simulink model "sparrow_albatros_spec_withgpio"  (R2021a)
settings: Solver=VariableStepDiscrete  StartTime=0.0  StopTime=100  RelTol=1e-3
undefined symbols (not defined in the file): pfb_coeff_gen_calc
libraries: xbsIndex_r4 x5582, casper_library_misc x33, casper_library_delays x28, xps_library x10, simulink x8, xbsReplacements_r4 x2
(part 31 of 80)

== system sparrow_albatros_spec_withgpio/fft_wideband_real/fft_biplex_real_4x/biplex_core/fft_stage_6 ==
  in1 : Inport
  in2 : Inport  Port=2
  of_in : Inport  Port=3
  sync : Inport  Port=4
  shift : Inport  Port=5
  butterfly_direct : Subsystem  AncestorBlock=casper_library_ffts/butterfly_direct  mask(butterfly_direct){n_inputs=1, biplex=on, FFTSize=FFTSize, Coeffs=[0 1 2 3 4 5 6 7 8 9 10 11 12 13 14 15 16 17 18 19 20 21 22 23 24 25 26 27 28 29 30 31], StepPeriod=5, coeff_bit_width=coeff_bit_width, input_bit_width=input_bit_width, bin_pt_in=bin_pt_in, downshift=off, async=off, floating_point=off, float_type=single, exp_width=8, frac_width=24, add_latency=add_latency, mult_latency=mult_latency, bram_latency=bram_latency, conv_latency=conv_latency, add_pipe_latency=0, mult_pipe_latency=0, quantization=Round  (unbiased: Even Values), overflow=Saturate, coeffs_bit_limit=coeffs_bit_limit, coeff_sharing=on, coeff_decimation=on, coeff_generation=off, cal_bits=1, n_bits_rotation=25, max_fanout=max_fanout, use_hdl=on, use_embedded=off, bitgrowth=on, hardcode_shifts=off, dsp48_adders=off}
      mask prompts: n_inputs "number inputs"; biplex "Used in biplex FFT"; FFTSize "Size of FFT: (2^? pts)"; Coeffs "Coefficients: (0 to 2^(FFTSize-1)-1)"; StepPeriod "Coefficient Step Period: (2^?)"; coeff_bit_width "Coefficient Bit Width"; input_bit_width "Input Bit Width"; bin_pt_in "Input binary point"; async "asynchronous operation"; floating_point "floating point"; float_type "float type"; exp_width "exponent width"; frac_width "fraction width"; add_latency "Add Latency"; mult_latency "Mult Latency"; bram_latency "BRAM Latency"; conv_latency "Convert latency"; add_pipe_latency "Add Pipeline Latency"; mult_pipe_latency "Mult Pipeline Latency"; quantization "Quantization Behavior"; overflow "Overflow Behavior"; coeffs_bit_limit "Number bits above which to store stage's coefficients in BRAM (2^? bits)"; coeff_sharing "BRAM sharing in coeff storage"; coeff_decimation "Store a fraction of coeff factors where useful"; coeff_generation "Generate coeffs with multipliers where useful"; cal_bits "Number calibration locations when generating coeffs (2^?)"; n_bits_rotation "Feedback rotation vector resolution"; max_fanout "Maximum fanout"; use_hdl "Use behavioural HDL for multipliers"; use_embedded "Use embedded multipliers"; bitgrowth "Bit growth instead of shifting"; hardcode_shifts "Hardcode shift schedule"; dsp48_adders "Use DSP48s for adders"
      mask help: FFT internal block.
      mask init: same as sparrow_albatros_spec_withgpio/fft_wideband_real/fft_direct/butterfly0_0
      settings: AttributesFormatString=twiddle_general
      mask Callback floating_point:
      | onoff = get_param(gcb, 'floating_point');
      | if strcmp(onoff,'on')
      |     enable_fixpt = 'off';
      |     set_param_state(gcb, 'float_type', 'on')
      | 
      |     f_type = get_param(gcb, 'float_type');
      |     if strcmp(f_type,'custom')
      |         set_param_state(gcb, 'exp_width', 'on')
      |         set_param_state(gcb, 'frac_width', 'on')
      |     else
      |         set_param_state(gcb, 'exp_width', 'off')
      |         set_param_state(gcb, 'frac_width', 'off')
      |     end
      | 
      | 
      | else
      |     enable_fixpt = 'on';
      |     set_param_state(gcb, 'float_type', 'off')
      |     set_param_state(gcb, 'exp_width', 'off')
      |     set_param_state(gcb, 'frac_width', 'off')
      | end
      | 
      | set_param_state(gcb, 'input_bit_width', enable_fixpt)
      | set_param_state(gcb, 'bin_pt_in', enable_fixpt)
      | set_param_state(gcb, 'coeff_bit_width', enable_fixpt)
      mask TypeOptions float_type: single | custom
      mask Callback float_type:
      | f_type = get_param(gcb, 'float_type');
      | if strcmp(f_type,'custom')
      |     set_param_state(gcb, 'exp_width', 'on')
      |     set_param_state(gcb, 'frac_width', 'on')
      | else
      |     set_param_state(gcb, 'exp_width', 'off')
      |     set_param_state(gcb, 'frac_width', 'off')
      | end
      mask TypeOptions quantization: Truncate | Round  (unbiased: +/- Inf) | Round  (unbiased: Even Values)
      mask TypeOptions overflow: Wrap | Saturate | Error
      mask Callback use_hdl:
      | % make mutually exclusive with use_embedded.
      | 
      | use_hdl = get_param(gcb, 'use_hdl');
      | if strcmp(use_hdl, 'on'),
      |     set_param_state(gcb, 'use_embedded', 'off');
      | else
      |     set_param_state(gcb, 'use_embedded', 'on');
      | end
      mask Callback use_embedded:
      | % make mutually exclusive with use_hdl.
      | 
      | use_hdl = get_param(gcb, 'use_embedded');
      | if strcmp(use_hdl, 'on'),
      |     set_param_state(gcb, 'use_hdl', 'off');
      | else
      |     set_param_state(gcb, 'use_hdl', 'on');
      | end
      mask Callback hardcode_shifts:
      | hardcode_shifts = get_param(gcb, 'hardcode_shifts');
      | set_param_state(gcb, 'downshift', hardcode_shifts);
      mask Callback dsp48_adders: %fft_callback_dsp48_adders(gcb);
      mask DialogControl ParameterTabVar0 Prompt: Basic
      mask DialogControl ParameterTabVar01 Prompt: Latency
      mask DialogControl ParameterTabVar012 Prompt: Implementation
  counter : xbsIndex_r4/Counter  cnt_type=Free Running  cnt_to=Inf  operation=Up  start_count=0  cnt_by_val=1  arith_type=Unsigned  n_bits=FFTSize-FFTStage+1  bin_pt=0  load_pin=off  rst=on  en=off  explicit_period=on  period=1  use_behavioral_HDL=off  implementation=Fabric  dbl_ovrd=off  block_type=counter
  delay0 : Subsystem  AncestorBlock=casper_library_bus/bus_delay  mask(bus_delay){n_bits=23, csp_latency=2^(FFTSize-FFTStage), cmplx=on, enable=off, reg_retiming=on, misc=off}
      mask prompts: n_bits "input bit widths"; csp_latency "latency"; cmplx "complex data"; enable "enable port"; reg_retiming "implement using behavioral HDL"; misc "misc support"
      mask help: Delay components of a bus
      mask init:
      | bus_delay_init(gcb, ...
      |     'enable', enable, ...
      |     'cmplx', cmplx, ...
      |     'n_bits', n_bits, ...
      |     'csp_latency', csp_latency, ...
      |     'reg_retiming', reg_retiming, ...
      |     'misc', misc);
  delay1 : Subsystem  AncestorBlock=casper_library_bus/bus_delay  mask(bus_delay){n_bits=23, csp_latency=2^(FFTSize-FFTStage), cmplx=on, enable=off, reg_retiming=on, misc=off}
      mask prompts: n_bits "input bit widths"; csp_latency "latency"; cmplx "complex data"; enable "enable port"; reg_retiming "implement using behavioral HDL"; misc "misc support"
      mask help: Delay components of a bus
      mask init:
      | bus_delay_init(gcb, ...
      |     'enable', enable, ...
      |     'cmplx', cmplx, ...
      |     'n_bits', n_bits, ...
      |     'csp_latency', csp_latency, ...
      |     'reg_retiming', reg_retiming, ...
      |     'misc', misc);
  din0 : xbsIndex_r4/Delay  rst=off  infoeditControl=Selection of Reset will increase slice count due to use of real FFs and instead of SRLs  en=off  latency=0  reg_retiming=on  dbl_ovrd=off  block_type=delay
  din2 : xbsIndex_r4/Delay  rst=off  infoeditControl=Selection of Reset will increase slice count due to use of real FFs and instead of SRLs  en=off  latency=0  reg_retiming=on  dbl_ovrd=off  block_type=delay
  dmux0 : xbsIndex_r4/Delay  rst=off  infoeditControl=Selection of Reset will increase slice count due to use of real FFs and instead of SRLs  en=off  latency=0  reg_retiming=on  dbl_ovrd=off  block_type=delay
  dmux1 : xbsIndex_r4/Delay  rst=off  infoeditControl=Selection of Reset will increase slice count due to use of real FFs and instead of SRLs  en=off  latency=0  reg_retiming=on  dbl_ovrd=off  block_type=delay
  dsync0 : xbsIndex_r4/Delay  rst=off  infoeditControl=Selection of Reset will increase slice count due to use of real FFs and instead of SRLs  en=off  latency=0  reg_retiming=on  dbl_ovrd=off  block_type=delay
  dsync1 : xbsIndex_r4/Delay  rst=off  infoeditControl=Selection of Reset will increase slice count due to use of real FFs and instead of SRLs  en=off  latency=1  reg_retiming=on  dbl_ovrd=off  block_type=delay
  logical1 : xbsIndex_r4/Logical  logical_function=OR  inputs=2  en=off  latency=1  precision=Full  arith_type=Unsigned  n_bits=16  bin_pt=0  align_bp=on  dbl_ovrd=off  block_type=logical
  mux0 : xbsIndex_r4/Mux  inputs=2  en=off  latency=1  precision=Full  arith_type=Unsigned  n_bits=16  bin_pt=14  quantization=Truncate  overflow=Wrap  dbl_ovrd=off  block_type=mux
  mux1 : xbsIndex_r4/Mux  inputs=2  en=off  latency=1  precision=Full  arith_type=Unsigned  n_bits=16  bin_pt=14  quantization=Truncate  overflow=Wrap  dbl_ovrd=off  block_type=mux
  slice0 : xbsIndex_r4/Slice  nbits=1  boolean_output=on  mode=Lower Bit Location + Width  bit1=-(FFTStage - 1)  base1=MSB of Input  bit0=FFTStage - 1  base0=LSB of Input  dbl_ovrd=off  block_type=slice
  slice1 : xbsIndex_r4/Slice  nbits=1  boolean_output=off  mode=Upper Bit Location + Width  bit1=0  base1=MSB of Input  bit0=0  base0=LSB of Input  dbl_ovrd=off  block_type=slice
  sync_delay : casper_library_delays/sync_delay  DelayLen=2^(FFTSize - FFTStage)
      settings: SourceProductName=CASPER DSP Blockset
  out1 : Outport
  out2 : Outport  Port=2
  of : Outport  Port=3
  sync_out : Outport  Port=4
  wires:
  in1/1 -> din0/1
  sync/1 -> dsync0/1
  counter/1 -> slice1/1
  slice1/1 -> mux1/1, mux0/1
  mux0/1 -> dmux0/1
  din0/1 -> mux1/2, mux0/3
  dsync0/1 -> dsync1/1, counter/1
  in2/1 -> din2/1
  din2/1 -> delay0/1(din)
  mux1/1 -> dmux1/1
  dmux1/1 -> delay1/1(din)
  delay0/1(dout) -> mux1/3, mux0/2
  dsync1/1 -> sync_delay/1
  shift/1 -> slice0/1
  dmux0/1 -> butterfly_direct/2(b)
  slice0/1 -> butterfly_direct/4(shift)
  delay1/1(dout) -> butterfly_direct/1(a)
  sync_delay/1 -> butterfly_direct/3(sync_in)
  of_in/1 -> logical1/2
  butterfly_direct/3(of) -> logical1/1
  butterfly_direct/1(a+bw) -> out1/1
  butterfly_direct/2(a-bw) -> out2/1
  logical1/1 -> of/1
  butterfly_direct/4(sync_out) -> sync_out/1

== system sparrow_albatros_spec_withgpio/fft_wideband_real/fft_biplex_real_4x/biplex_core/fft_stage_7 ==
  in1 : Inport
  in2 : Inport  Port=2
  of_in : Inport  Port=3
  sync : Inport  Port=4
  shift : Inport  Port=5
  butterfly_direct : Subsystem  AncestorBlock=casper_library_ffts/butterfly_direct  mask(butterfly_direct){n_inputs=1, biplex=on, FFTSize=FFTSize, Coeffs=[0 1 2 3 4 5 6 7 8 9 10 11 12 13 14 15 16 17 18 19 20 21 22 23 24 25 26 27 28 29 30 31 32 33 34 35 36 37 38 39 40 41 42 43 44 45 46 47 48 49 50 51 52 53 54 55 56 57 58 59 60 61 62 63], StepPeriod=4, coeff_bit_width=coeff_bit_width, input_bit_width=input_bit_width, bin_pt_in=bin_pt_in, downshift=off, async=off, floating_point=off, float_type=single, exp_width=8, frac_width=24, add_latency=add_latency, mult_latency=mult_latency, bram_latency=bram_latency, conv_latency=conv_latency, add_pipe_latency=0, mult_pipe_latency=0, quantization=Round  (unbiased: Even Values), overflow=Saturate, coeffs_bit_limit=coeffs_bit_limit, coeff_sharing=on, coeff_decimation=on, coeff_generation=off, cal_bits=1, n_bits_rotation=25, max_fanout=max_fanout, use_hdl=on, use_embedded=off, bitgrowth=off, hardcode_shifts=off, dsp48_adders=off}
      mask prompts: n_inputs "number inputs"; biplex "Used in biplex FFT"; FFTSize "Size of FFT: (2^? pts)"; Coeffs "Coefficients: (0 to 2^(FFTSize-1)-1)"; StepPeriod "Coefficient Step Period: (2^?)"; coeff_bit_width "Coefficient Bit Width"; input_bit_width "Input Bit Width"; bin_pt_in "Input binary point"; async "asynchronous operation"; floating_point "floating point"; float_type "float type"; exp_width "exponent width"; frac_width "fraction width"; add_latency "Add Latency"; mult_latency "Mult Latency"; bram_latency "BRAM Latency"; conv_latency "Convert latency"; add_pipe_latency "Add Pipeline Latency"; mult_pipe_latency "Mult Pipeline Latency"; quantization "Quantization Behavior"; overflow "Overflow Behavior"; coeffs_bit_limit "Number bits above which to store stage's coefficients in BRAM (2^? bits)"; coeff_sharing "BRAM sharing in coeff storage"; coeff_decimation "Store a fraction of coeff factors where useful"; coeff_generation "Generate coeffs with multipliers where useful"; cal_bits "Number calibration locations when generating coeffs (2^?)"; n_bits_rotation "Feedback rotation vector resolution"; max_fanout "Maximum fanout"; use_hdl "Use behavioural HDL for multipliers"; use_embedded "Use embedded multipliers"; bitgrowth "Bit growth instead of shifting"; hardcode_shifts "Hardcode shift schedule"; dsp48_adders "Use DSP48s for adders"
      mask help: FFT internal block.
      mask init: same as sparrow_albatros_spec_withgpio/fft_wideband_real/fft_direct/butterfly0_0
      settings: AttributesFormatString=twiddle_general
      mask Callback floating_point:
      | onoff = get_param(gcb, 'floating_point');
      | if strcmp(onoff,'on')
      |     enable_fixpt = 'off';
      |     set_param_state(gcb, 'float_type', 'on')
      | 
      |     f_type = get_param(gcb, 'float_type');
      |     if strcmp(f_type,'custom')
      |         set_param_state(gcb, 'exp_width', 'on')
      |         set_param_state(gcb, 'frac_width', 'on')
      |     else
      |         set_param_state(gcb, 'exp_width', 'off')
      |         set_param_state(gcb, 'frac_width', 'off')
      |     end
      | 
      | 
      | else
      |     enable_fixpt = 'on';
      |     set_param_state(gcb, 'float_type', 'off')
      |     set_param_state(gcb, 'exp_width', 'off')
      |     set_param_state(gcb, 'frac_width', 'off')
      | end
      | 
      | set_param_state(gcb, 'input_bit_width', enable_fixpt)
      | set_param_state(gcb, 'bin_pt_in', enable_fixpt)
      | set_param_state(gcb, 'coeff_bit_width', enable_fixpt)
      mask TypeOptions float_type: single | custom
      mask Callback float_type:
      | f_type = get_param(gcb, 'float_type');
      | if strcmp(f_type,'custom')
      |     set_param_state(gcb, 'exp_width', 'on')
      |     set_param_state(gcb, 'frac_width', 'on')
      | else
      |     set_param_state(gcb, 'exp_width', 'off')
      |     set_param_state(gcb, 'frac_width', 'off')
      | end
      mask TypeOptions quantization: Truncate | Round  (unbiased: +/- Inf) | Round  (unbiased: Even Values)
      mask TypeOptions overflow: Wrap | Saturate | Error
      mask Callback use_hdl:
      | % make mutually exclusive with use_embedded.
      | 
      | use_hdl = get_param(gcb, 'use_hdl');
      | if strcmp(use_hdl, 'on'),
      |     set_param_state(gcb, 'use_embedded', 'off');
      | else
      |     set_param_state(gcb, 'use_embedded', 'on');
      | end
      mask Callback use_embedded:
      | % make mutually exclusive with use_hdl.
      | 
      | use_hdl = get_param(gcb, 'use_embedded');
      | if strcmp(use_hdl, 'on'),
      |     set_param_state(gcb, 'use_hdl', 'off');
      | else
      |     set_param_state(gcb, 'use_hdl', 'on');
      | end
      mask Callback hardcode_shifts:
      | hardcode_shifts = get_param(gcb, 'hardcode_shifts');
      | set_param_state(gcb, 'downshift', hardcode_shifts);
      mask Callback dsp48_adders: %fft_callback_dsp48_adders(gcb);
      mask DialogControl ParameterTabVar0 Prompt: Basic
      mask DialogControl ParameterTabVar01 Prompt: Latency
      mask DialogControl ParameterTabVar012 Prompt: Implementation
  counter : xbsIndex_r4/Counter  cnt_type=Free Running  cnt_to=Inf  operation=Up  start_count=0  cnt_by_val=1  arith_type=Unsigned  n_bits=FFTSize-FFTStage+1  bin_pt=0  load_pin=off  rst=on  en=off  explicit_period=on  period=1  use_behavioral_HDL=off  implementation=Fabric  dbl_ovrd=off  block_type=counter
  delay0 : Subsystem  AncestorBlock=casper_library_bus/bus_delay  mask(bus_delay){n_bits=24, csp_latency=2^(FFTSize-FFTStage), cmplx=on, enable=off, reg_retiming=on, misc=off}
      mask prompts: n_bits "input bit widths"; csp_latency "latency"; cmplx "complex data"; enable "enable port"; reg_retiming "implement using behavioral HDL"; misc "misc support"
      mask help: Delay components of a bus
      mask init:
      | bus_delay_init(gcb, ...
      |     'enable', enable, ...
      |     'cmplx', cmplx, ...
      |     'n_bits', n_bits, ...
      |     'csp_latency', csp_latency, ...
      |     'reg_retiming', reg_retiming, ...
      |     'misc', misc);
  delay1 : Subsystem  AncestorBlock=casper_library_bus/bus_delay  mask(bus_delay){n_bits=24, csp_latency=2^(FFTSize-FFTStage), cmplx=on, enable=off, reg_retiming=on, misc=off}
      mask prompts: n_bits "input bit widths"; csp_latency "latency"; cmplx "complex data"; enable "enable port"; reg_retiming "implement using behavioral HDL"; misc "misc support"
      mask help: Delay components of a bus
      mask init:
      | bus_delay_init(gcb, ...
      |     'enable', enable, ...
      |     'cmplx', cmplx, ...
      |     'n_bits', n_bits, ...
      |     'csp_latency', csp_latency, ...
      |     'reg_retiming', reg_retiming, ...
      |     'misc', misc);
  din0 : xbsIndex_r4/Delay  rst=off  infoeditControl=Selection of Reset will increase slice count due to use of real FFs and instead of SRLs  en=off  latency=0  reg_retiming=on  dbl_ovrd=off  block_type=delay
  din2 : xbsIndex_r4/Delay  rst=off  infoeditControl=Selection of Reset will increase slice count due to use of real FFs and instead of SRLs  en=off  latency=0  reg_retiming=on  dbl_ovrd=off  block_type=delay
  dmux0 : xbsIndex_r4/Delay  rst=off  infoeditControl=Selection of Reset will increase slice count due to use of real FFs and instead of SRLs  en=off  latency=0  reg_retiming=on  dbl_ovrd=off  block_type=delay
  dmux1 : xbsIndex_r4/Delay  rst=off  infoeditControl=Selection of Reset will increase slice count due to use of real FFs and instead of SRLs  en=off  latency=0  reg_retiming=on  dbl_ovrd=off  block_type=delay
  dsync0 : xbsIndex_r4/Delay  rst=off  infoeditControl=Selection of Reset will increase slice count due to use of real FFs and instead of SRLs  en=off  latency=0  reg_retiming=on  dbl_ovrd=off  block_type=delay
  dsync1 : xbsIndex_r4/Delay  rst=off  infoeditControl=Selection of Reset will increase slice count due to use of real FFs and instead of SRLs  en=off  latency=1  reg_retiming=on  dbl_ovrd=off  block_type=delay
  logical1 : xbsIndex_r4/Logical  logical_function=OR  inputs=2  en=off  latency=1  precision=Full  arith_type=Unsigned  n_bits=16  bin_pt=0  align_bp=on  dbl_ovrd=off  block_type=logical
  mux0 : xbsIndex_r4/Mux  inputs=2  en=off  latency=1  precision=Full  arith_type=Unsigned  n_bits=16  bin_pt=14  quantization=Truncate  overflow=Wrap  dbl_ovrd=off  block_type=mux
  mux1 : xbsIndex_r4/Mux  inputs=2  en=off  latency=1  precision=Full  arith_type=Unsigned  n_bits=16  bin_pt=14  quantization=Truncate  overflow=Wrap  dbl_ovrd=off  block_type=mux
  slice0 : xbsIndex_r4/Slice  nbits=1  boolean_output=on  mode=Lower Bit Location + Width  bit1=-(FFTStage - 1)  base1=MSB of Input  bit0=FFTStage - 1  base0=LSB of Input  dbl_ovrd=off  block_type=slice
  slice1 : xbsIndex_r4/Slice  nbits=1  boolean_output=off  mode=Upper Bit Location + Width  bit1=0  base1=MSB of Input  bit0=0  base0=LSB of Input  dbl_ovrd=off  block_type=slice
  sync_delay : casper_library_delays/sync_delay  DelayLen=2^(FFTSize - FFTStage)
      settings: SourceProductName=CASPER DSP Blockset
  out1 : Outport
  out2 : Outport  Port=2
  of : Outport  Port=3
  sync_out : Outport  Port=4
  wires:
  in1/1 -> din0/1
  sync/1 -> dsync0/1
  counter/1 -> slice1/1
  slice1/1 -> mux1/1, mux0/1
  mux0/1 -> dmux0/1
  din0/1 -> mux1/2, mux0/3
  dsync0/1 -> dsync1/1, counter/1
  in2/1 -> din2/1
  din2/1 -> delay0/1(din)
  mux1/1 -> dmux1/1
  dmux1/1 -> delay1/1(din)
  delay0/1(dout) -> mux1/3, mux0/2
  dsync1/1 -> sync_delay/1
  shift/1 -> slice0/1
  dmux0/1 -> butterfly_direct/2(b)
  slice0/1 -> butterfly_direct/4(shift)
  delay1/1(dout) -> butterfly_direct/1(a)
  sync_delay/1 -> butterfly_direct/3(sync_in)
  of_in/1 -> logical1/2
  butterfly_direct/3(of) -> logical1/1
  butterfly_direct/1(a+bw) -> out1/1
  butterfly_direct/2(a-bw) -> out2/1
  logical1/1 -> of/1
  butterfly_direct/4(sync_out) -> sync_out/1

== system sparrow_albatros_spec_withgpio/fft_wideband_real/fft_biplex_real_4x/biplex_core/fft_stage_8 ==
  in1 : Inport
  in2 : Inport  Port=2
  of_in : Inport  Port=3
  sync : Inport  Port=4
  shift : Inport  Port=5
  butterfly_direct : Subsystem  AncestorBlock=casper_library_ffts/butterfly_direct  mask(butterfly_direct){n_inputs=1, biplex=on, FFTSize=FFTSize, Coeffs=[0 1 2 3 4 5 6 7 8 9 10 11 12 13 14 15 16 17 18 19 20 21 22 23 24 25 26 27 28 29 30 31 32 33 34 35 36 37 38 39 40 41 42 43 44 45 46 47 48 49 50 51 52 53 54 55 56 57 58 59 60 61 62 63 64 65 66 67 68 69 70 71 72 73 74 75 76 77 78 79 80 81 82 83 84 85 86 87 88 89 90 91 92 93 94 95 96 97 98 99 100 101 102 103 104 105 106 107 108 109 110 111 112 113 114 115 116 117 118 119 120 121 122 123 124 125 126 127], StepPeriod=3, coeff_bit_width=coeff_bit_width, input_bit_width=input_bit_width, bin_pt_in=bin_pt_in, downshift=off, async=off, floating_point=off, float_type=single, exp_width=8, frac_width=24, add_latency=add_latency, mult_latency=mult_latency, bram_latency=bram_latency, conv_latency=conv_latency, add_pipe_latency=0, mult_pipe_latency=0, quantization=Round  (unbiased: Even Values), overflow=Saturate, coeffs_bit_limit=coeffs_bit_limit, coeff_sharing=on, coeff_decimation=on, coeff_generation=off, cal_bits=1, n_bits_rotation=25, max_fanout=max_fanout, use_hdl=on, use_embedded=off, bitgrowth=off, hardcode_shifts=off, dsp48_adders=off}
      mask prompts: n_inputs "number inputs"; biplex "Used in biplex FFT"; FFTSize "Size of FFT: (2^? pts)"; Coeffs "Coefficients: (0 to 2^(FFTSize-1)-1)"; StepPeriod "Coefficient Step Period: (2^?)"; coeff_bit_width "Coefficient Bit Width"; input_bit_width "Input Bit Width"; bin_pt_in "Input binary point"; async "asynchronous operation"; floating_point "floating point"; float_type "float type"; exp_width "exponent width"; frac_width "fraction width"; add_latency "Add Latency"; mult_latency "Mult Latency"; bram_latency "BRAM Latency"; conv_latency "Convert latency"; add_pipe_latency "Add Pipeline Latency"; mult_pipe_latency "Mult Pipeline Latency"; quantization "Quantization Behavior"; overflow "Overflow Behavior"; coeffs_bit_limit "Number bits above which to store stage's coefficients in BRAM (2^? bits)"; coeff_sharing "BRAM sharing in coeff storage"; coeff_decimation "Store a fraction of coeff factors where useful"; coeff_generation "Generate coeffs with multipliers where useful"; cal_bits "Number calibration locations when generating coeffs (2^?)"; n_bits_rotation "Feedback rotation vector resolution"; max_fanout "Maximum fanout"; use_hdl "Use behavioural HDL for multipliers"; use_embedded "Use embedded multipliers"; bitgrowth "Bit growth instead of shifting"; hardcode_shifts "Hardcode shift schedule"; dsp48_adders "Use DSP48s for adders"
      mask help: FFT internal block.
      mask init: same as sparrow_albatros_spec_withgpio/fft_wideband_real/fft_direct/butterfly0_0
      settings: AttributesFormatString=twiddle_general
      mask Callback floating_point:
      | onoff = get_param(gcb, 'floating_point');
      | if strcmp(onoff,'on')
      |     enable_fixpt = 'off';
      |     set_param_state(gcb, 'float_type', 'on')
      | 
      |     f_type = get_param(gcb, 'float_type');
      |     if strcmp(f_type,'custom')
      |         set_param_state(gcb, 'exp_width', 'on')
      |         set_param_state(gcb, 'frac_width', 'on')
      |     else
      |         set_param_state(gcb, 'exp_width', 'off')
      |         set_param_state(gcb, 'frac_width', 'off')
      |     end
      | 
      | 
      | else
      |     enable_fixpt = 'on';
      |     set_param_state(gcb, 'float_type', 'off')
      |     set_param_state(gcb, 'exp_width', 'off')
      |     set_param_state(gcb, 'frac_width', 'off')
      | end
      | 
      | set_param_state(gcb, 'input_bit_width', enable_fixpt)
      | set_param_state(gcb, 'bin_pt_in', enable_fixpt)
      | set_param_state(gcb, 'coeff_bit_width', enable_fixpt)
      mask TypeOptions float_type: single | custom
      mask Callback float_type:
      | f_type = get_param(gcb, 'float_type');
      | if strcmp(f_type,'custom')
      |     set_param_state(gcb, 'exp_width', 'on')
      |     set_param_state(gcb, 'frac_width', 'on')
      | else
      |     set_param_state(gcb, 'exp_width', 'off')
      |     set_param_state(gcb, 'frac_width', 'off')
      | end
      mask TypeOptions quantization: Truncate | Round  (unbiased: +/- Inf) | Round  (unbiased: Even Values)
      mask TypeOptions overflow: Wrap | Saturate | Error
      mask Callback use_hdl:
      | % make mutually exclusive with use_embedded.
      | 
      | use_hdl = get_param(gcb, 'use_hdl');
      | if strcmp(use_hdl, 'on'),
      |     set_param_state(gcb, 'use_embedded', 'off');
      | else
      |     set_param_state(gcb, 'use_embedded', 'on');
      | end
      mask Callback use_embedded:
      | % make mutually exclusive with use_hdl.
      | 
      | use_hdl = get_param(gcb, 'use_embedded');
      | if strcmp(use_hdl, 'on'),
      |     set_param_state(gcb, 'use_hdl', 'off');
      | else
      |     set_param_state(gcb, 'use_hdl', 'on');
      | end
      mask Callback hardcode_shifts:
      | hardcode_shifts = get_param(gcb, 'hardcode_shifts');
      | set_param_state(gcb, 'downshift', hardcode_shifts);
      mask Callback dsp48_adders: %fft_callback_dsp48_adders(gcb);
      mask DialogControl ParameterTabVar0 Prompt: Basic
      mask DialogControl ParameterTabVar01 Prompt: Latency
      mask DialogControl ParameterTabVar012 Prompt: Implementation
  counter : xbsIndex_r4/Counter  cnt_type=Free Running  cnt_to=Inf  operation=Up  start_count=0  cnt_by_val=1  arith_type=Unsigned  n_bits=FFTSize-FFTStage+1  bin_pt=0  load_pin=off  rst=on  en=off  explicit_period=on  period=1  use_behavioral_HDL=off  implementation=Fabric  dbl_ovrd=off  block_type=counter
  delay0 : Subsystem  AncestorBlock=casper_library_bus/bus_delay  mask(bus_delay){n_bits=24, csp_latency=2^(FFTSize-FFTStage), cmplx=on, enable=off, reg_retiming=on, misc=off}
      mask prompts: n_bits "input bit widths"; csp_latency "latency"; cmplx "complex data"; enable "enable port"; reg_retiming "implement using behavioral HDL"; misc "misc support"
      mask help: Delay components of a bus
      mask init:
      | bus_delay_init(gcb, ...
      |     'enable', enable, ...
      |     'cmplx', cmplx, ...
      |     'n_bits', n_bits, ...
      |     'csp_latency', csp_latency, ...
      |     'reg_retiming', reg_retiming, ...
      |     'misc', misc);
  delay1 : Subsystem  AncestorBlock=casper_library_bus/bus_delay  mask(bus_delay){n_bits=24, csp_latency=2^(FFTSize-FFTStage), cmplx=on, enable=off, reg_retiming=on, misc=off}
      mask prompts: n_bits "input bit widths"; csp_latency "latency"; cmplx "complex data"; enable "enable port"; reg_retiming "implement using behavioral HDL"; misc "misc support"
      mask help: Delay components of a bus
      mask init:
      | bus_delay_init(gcb, ...
      |     'enable', enable, ...
      |     'cmplx', cmplx, ...
      |     'n_bits', n_bits, ...
      |     'csp_latency', csp_latency, ...
      |     'reg_retiming', reg_retiming, ...
      |     'misc', misc);
  din0 : xbsIndex_r4/Delay  rst=off  infoeditControl=Selection of Reset will increase slice count due to use of real FFs and instead of SRLs  en=off  latency=0  reg_retiming=on  dbl_ovrd=off  block_type=delay
  din2 : xbsIndex_r4/Delay  rst=off  infoeditControl=Selection of Reset will increase slice count due to use of real FFs and instead of SRLs  en=off  latency=0  reg_retiming=on  dbl_ovrd=off  block_type=delay
  dmux0 : xbsIndex_r4/Delay  rst=off  infoeditControl=Selection of Reset will increase slice count due to use of real FFs and instead of SRLs  en=off  latency=0  reg_retiming=on  dbl_ovrd=off  block_type=delay
  dmux1 : xbsIndex_r4/Delay  rst=off  infoeditControl=Selection of Reset will increase slice count due to use of real FFs and instead of SRLs  en=off  latency=0  reg_retiming=on  dbl_ovrd=off  block_type=delay
  dsync0 : xbsIndex_r4/Delay  rst=off  infoeditControl=Selection of Reset will increase slice count due to use of real FFs and instead of SRLs  en=off  latency=0  reg_retiming=on  dbl_ovrd=off  block_type=delay
  dsync1 : xbsIndex_r4/Delay  rst=off  infoeditControl=Selection of Reset will increase slice count due to use of real FFs and instead of SRLs  en=off  latency=1  reg_retiming=on  dbl_ovrd=off  block_type=delay
  logical1 : xbsIndex_r4/Logical  logical_function=OR  inputs=2  en=off  latency=1  precision=Full  arith_type=Unsigned  n_bits=16  bin_pt=0  align_bp=on  dbl_ovrd=off  block_type=logical
  mux0 : xbsIndex_r4/Mux  inputs=2  en=off  latency=1  precision=Full  arith_type=Unsigned  n_bits=16  bin_pt=14  quantization=Truncate  overflow=Wrap  dbl_ovrd=off  block_type=mux
  mux1 : xbsIndex_r4/Mux  inputs=2  en=off  latency=1  precision=Full  arith_type=Unsigned  n_bits=16  bin_pt=14  quantization=Truncate  overflow=Wrap  dbl_ovrd=off  block_type=mux
  slice0 : xbsIndex_r4/Slice  nbits=1  boolean_output=on  mode=Lower Bit Location + Width  bit1=-(FFTStage - 1)  base1=MSB of Input  bit0=FFTStage - 1  base0=LSB of Input  dbl_ovrd=off  block_type=slice
  slice1 : xbsIndex_r4/Slice  nbits=1  boolean_output=off  mode=Upper Bit Location + Width  bit1=0  base1=MSB of Input  bit0=0  base0=LSB of Input  dbl_ovrd=off  block_type=slice
  sync_delay : casper_library_delays/sync_delay  DelayLen=2^(FFTSize - FFTStage)
      settings: SourceProductName=CASPER DSP Blockset
  out1 : Outport
  out2 : Outport  Port=2
  of : Outport  Port=3
  sync_out : Outport  Port=4
  wires:
  in1/1 -> din0/1
  sync/1 -> dsync0/1
  counter/1 -> slice1/1
  slice1/1 -> mux1/1, mux0/1
  mux0/1 -> dmux0/1
  din0/1 -> mux1/2, mux0/3
  dsync0/1 -> dsync1/1, counter/1
  in2/1 -> din2/1
  din2/1 -> delay0/1(din)
  mux1/1 -> dmux1/1
  dmux1/1 -> delay1/1(din)
  delay0/1(dout) -> mux1/3, mux0/2
  dsync1/1 -> sync_delay/1
  shift/1 -> slice0/1
  dmux0/1 -> butterfly_direct/2(b)
  slice0/1 -> butterfly_direct/4(shift)
  delay1/1(dout) -> butterfly_direct/1(a)
  sync_delay/1 -> butterfly_direct/3(sync_in)
  of_in/1 -> logical1/2
  butterfly_direct/3(of) -> logical1/1
  butterfly_direct/1(a+bw) -> out1/1
  butterfly_direct/2(a-bw) -> out2/1
  logical1/1 -> of/1
  butterfly_direct/4(sync_out) -> sync_out/1

== system sparrow_albatros_spec_withgpio/fft_wideband_real/fft_biplex_real_4x/biplex_core/fft_stage_9 ==
  in1 : Inport
  in2 : Inport  Port=2
  of_in : Inport  Port=3
  sync : Inport  Port=4
  shift : Inport  Port=5
  butterfly_direct : Subsystem  AncestorBlock=casper_library_ffts/butterfly_direct  mask(butterfly_direct){n_inputs=1, biplex=on, FFTSize=FFTSize, Coeffs=[0 1 2 3 4 5 6 7 8 9 10 11 12 13 14 15 16 17 18 19 20 21 22 23 24 25 26 27 28 29 30 31 32 33 34 35 36 37 38 39 40 41 42 43 44 45 46 47 48 49 50 51 52 53 54 55 56 57 58 59 60 61 62 63 64 65 66 67 68 69 70 71 72 73 74 75 76 77 78 79 80 81 82 83 84 85 86 87 88 89 90 91 92 93 94 95 96 97 98 99 100 101 102 103 104 105 106 107 108 109 110 111 112 113 114 115 116 117 118 119 120 121 122 123 124 125 126 127 128 129 130 131 132 133 134 135 136 137 138 139 140 141 142 143 144 145 146 147 148 149 150 151 152 153 154 155 156 157 158 159 160 161 162 163 164 165 166 167 168 169 170 171 172 173 174 175 176 177 178 179 180 181 182 183 184 185 186 187 188 189 190 191 192 193 194 195 196 197 198 199 200 201 202 203 204 205 206 207 208 209 210 211 212 213 214 215 216 217 218 219 220 221 222 223 224 225 226 227 228 229 230 231 232 233 234 235 236 237 238 239 240 241 242 243 244 245 246 247 248 249 250 251 252 253 254 255], StepPeriod=2, coeff_bit_width=coeff_bit_width, input_bit_width=input_bit_width, bin_pt_in=bin_pt_in, downshift=off, async=off, floating_point=off, float_type=single, exp_width=8, frac_width=24, add_latency=add_latency, mult_latency=mult_latency, bram_latency=bram_latency, conv_latency=conv_latency, add_pipe_latency=0, mult_pipe_latency=0, quantization=Round  (unbiased: Even Values), overflow=Saturate, coeffs_bit_limit=coeffs_bit_limit, coeff_sharing=on, coeff_decimation=on, coeff_generation=off, cal_bits=1, n_bits_rotation=25, max_fanout=max_fanout, use_hdl=on, use_embedded=off, bitgrowth=off, hardcode_shifts=off, dsp48_adders=off}
      mask prompts: n_inputs "number inputs"; biplex "Used in biplex FFT"; FFTSize "Size of FFT: (2^? pts)"; Coeffs "Coefficients: (0 to 2^(FFTSize-1)-1)"; StepPeriod "Coefficient Step Period: (2^?)"; coeff_bit_width "Coefficient Bit Width"; input_bit_width "Input Bit Width"; bin_pt_in "Input binary point"; async "asynchronous operation"; floating_point "floating point"; float_type "float type"; exp_width "exponent width"; frac_width "fraction width"; add_latency "Add Latency"; mult_latency "Mult Latency"; bram_latency "BRAM Latency"; conv_latency "Convert latency"; add_pipe_latency "Add Pipeline Latency"; mult_pipe_latency "Mult Pipeline Latency"; quantization "Quantization Behavior"; overflow "Overflow Behavior"; coeffs_bit_limit "Number bits above which to store stage's coefficients in BRAM (2^? bits)"; coeff_sharing "BRAM sharing in coeff storage"; coeff_decimation "Store a fraction of coeff factors where useful"; coeff_generation "Generate coeffs with multipliers where useful"; cal_bits "Number calibration locations when generating coeffs (2^?)"; n_bits_rotation "Feedback rotation vector resolution"; max_fanout "Maximum fanout"; use_hdl "Use behavioural HDL for multipliers"; use_embedded "Use embedded multipliers"; bitgrowth "Bit growth instead of shifting"; hardcode_shifts "Hardcode shift schedule"; dsp48_adders "Use DSP48s for adders"
      mask help: FFT internal block.
      mask init: same as sparrow_albatros_spec_withgpio/fft_wideband_real/fft_direct/butterfly0_0
      settings: AttributesFormatString=twiddle_general
      mask Callback floating_point:
      | onoff = get_param(gcb, 'floating_point');
      | if strcmp(onoff,'on')
      |     enable_fixpt = 'off';
      |     set_param_state(gcb, 'float_type', 'on')
      | 
      |     f_type = get_param(gcb, 'float_type');
      |     if strcmp(f_type,'custom')
      |         set_param_state(gcb, 'exp_width', 'on')
      |         set_param_state(gcb, 'frac_width', 'on')
      |     else
      |         set_param_state(gcb, 'exp_width', 'off')
      |         set_param_state(gcb, 'frac_width', 'off')
      |     end
      | 
      | 
      | else
      |     enable_fixpt = 'on';
      |     set_param_state(gcb, 'float_type', 'off')
      |     set_param_state(gcb, 'exp_width', 'off')
      |     set_param_state(gcb, 'frac_width', 'off')
      | end
      | 
      | set_param_state(gcb, 'input_bit_width', enable_fixpt)
      | set_param_state(gcb, 'bin_pt_in', enable_fixpt)
      | set_param_state(gcb, 'coeff_bit_width', enable_fixpt)
      mask TypeOptions float_type: single | custom
      mask Callback float_type:
      | f_type = get_param(gcb, 'float_type');
      | if strcmp(f_type,'custom')
      |     set_param_state(gcb, 'exp_width', 'on')
      |     set_param_state(gcb, 'frac_width', 'on')
      | else
      |     set_param_state(gcb, 'exp_width', 'off')
      |     set_param_state(gcb, 'frac_width', 'off')
      | end
      mask TypeOptions quantization: Truncate | Round  (unbiased: +/- Inf) | Round  (unbiased: Even Values)
      mask TypeOptions overflow: Wrap | Saturate | Error
      mask Callback use_hdl:
      | % make mutually exclusive with use_embedded.
      | 
      | use_hdl = get_param(gcb, 'use_hdl');
      | if strcmp(use_hdl, 'on'),
      |     set_param_state(gcb, 'use_embedded', 'off');
      | else
      |     set_param_state(gcb, 'use_embedded', 'on');
      | end
      mask Callback use_embedded:
      | % make mutually exclusive with use_hdl.
      | 
      | use_hdl = get_param(gcb, 'use_embedded');
      | if strcmp(use_hdl, 'on'),
      |     set_param_state(gcb, 'use_hdl', 'off');
      | else
      |     set_param_state(gcb, 'use_hdl', 'on');
      | end
      mask Callback hardcode_shifts:
      | hardcode_shifts = get_param(gcb, 'hardcode_shifts');
      | set_param_state(gcb, 'downshift', hardcode_shifts);
      mask Callback dsp48_adders: %fft_callback_dsp48_adders(gcb);
      mask DialogControl ParameterTabVar0 Prompt: Basic
      mask DialogControl ParameterTabVar01 Prompt: Latency
      mask DialogControl ParameterTabVar012 Prompt: Implementation
  counter : xbsIndex_r4/Counter  cnt_type=Free Running  cnt_to=Inf  operation=Up  start_count=0  cnt_by_val=1  arith_type=Unsigned  n_bits=FFTSize-FFTStage+1  bin_pt=0  load_pin=off  rst=on  en=off  explicit_period=on  period=1  use_behavioral_HDL=off  implementation=Fabric  dbl_ovrd=off  block_type=counter
  delay0 : Subsystem  AncestorBlock=casper_library_bus/bus_delay  mask(bus_delay){n_bits=24, csp_latency=2^(FFTSize-FFTStage), cmplx=on, enable=off, reg_retiming=on, misc=off}
      mask prompts: n_bits "input bit widths"; csp_latency "latency"; cmplx "complex data"; enable "enable port"; reg_retiming "implement using behavioral HDL"; misc "misc support"
      mask help: Delay components of a bus
      mask init:
      | bus_delay_init(gcb, ...
      |     'enable', enable, ...
      |     'cmplx', cmplx, ...
      |     'n_bits', n_bits, ...
      |     'csp_latency', csp_latency, ...
      |     'reg_retiming', reg_retiming, ...
      |     'misc', misc);
  delay1 : Subsystem  AncestorBlock=casper_library_bus/bus_delay  mask(bus_delay){n_bits=24, csp_latency=2^(FFTSize-FFTStage), cmplx=on, enable=off, reg_retiming=on, misc=off}
      mask prompts: n_bits "input bit widths"; csp_latency "latency"; cmplx "complex data"; enable "enable port"; reg_retiming "implement using behavioral HDL"; misc "misc support"
      mask help: Delay components of a bus
      mask init:
      | bus_delay_init(gcb, ...
      |     'enable', enable, ...
      |     'cmplx', cmplx, ...
      |     'n_bits', n_bits, ...
      |     'csp_latency', csp_latency, ...
      |     'reg_retiming', reg_retiming, ...
      |     'misc', misc);
  din0 : xbsIndex_r4/Delay  rst=off  infoeditControl=Selection of Reset will increase slice count due to use of real FFs and instead of SRLs  en=off  latency=0  reg_retiming=on  dbl_ovrd=off  block_type=delay
  din2 : xbsIndex_r4/Delay  rst=off  infoeditControl=Selection of Reset will increase slice count due to use of real FFs and instead of SRLs  en=off  latency=0  reg_retiming=on  dbl_ovrd=off  block_type=delay
  dmux0 : xbsIndex_r4/Delay  rst=off  infoeditControl=Selection of Reset will increase slice count due to use of real FFs and instead of SRLs  en=off  latency=0  reg_retiming=on  dbl_ovrd=off  block_type=delay
  dmux1 : xbsIndex_r4/Delay  rst=off  infoeditControl=Selection of Reset will increase slice count due to use of real FFs and instead of SRLs  en=off  latency=0  reg_retiming=on  dbl_ovrd=off  block_type=delay
  dsync0 : xbsIndex_r4/Delay  rst=off  infoeditControl=Selection of Reset will increase slice count due to use of real FFs and instead of SRLs  en=off  latency=0  reg_retiming=on  dbl_ovrd=off  block_type=delay
  dsync1 : xbsIndex_r4/Delay  rst=off  infoeditControl=Selection of Reset will increase slice count due to use of real FFs and instead of SRLs  en=off  latency=1  reg_retiming=on  dbl_ovrd=off  block_type=delay
  logical1 : xbsIndex_r4/Logical  logical_function=OR  inputs=2  en=off  latency=1  precision=Full  arith_type=Unsigned  n_bits=16  bin_pt=0  align_bp=on  dbl_ovrd=off  block_type=logical
  mux0 : xbsIndex_r4/Mux  inputs=2  en=off  latency=1  precision=Full  arith_type=Unsigned  n_bits=16  bin_pt=14  quantization=Truncate  overflow=Wrap  dbl_ovrd=off  block_type=mux
  mux1 : xbsIndex_r4/Mux  inputs=2  en=off  latency=1  precision=Full  arith_type=Unsigned  n_bits=16  bin_pt=14  quantization=Truncate  overflow=Wrap  dbl_ovrd=off  block_type=mux
  slice0 : xbsIndex_r4/Slice  nbits=1  boolean_output=on  mode=Lower Bit Location + Width  bit1=-(FFTStage - 1)  base1=MSB of Input  bit0=FFTStage - 1  base0=LSB of Input  dbl_ovrd=off  block_type=slice
  slice1 : xbsIndex_r4/Slice  nbits=1  boolean_output=off  mode=Upper Bit Location + Width  bit1=0  base1=MSB of Input  bit0=0  base0=LSB of Input  dbl_ovrd=off  block_type=slice
  sync_delay : casper_library_delays/sync_delay  DelayLen=2^(FFTSize - FFTStage)
      settings: SourceProductName=CASPER DSP Blockset
  out1 : Outport
  out2 : Outport  Port=2
  of : Outport  Port=3
  sync_out : Outport  Port=4
  wires:
  in1/1 -> din0/1
  sync/1 -> dsync0/1
  counter/1 -> slice1/1
  slice1/1 -> mux1/1, mux0/1
  mux0/1 -> dmux0/1
  din0/1 -> mux1/2, mux0/3
  dsync0/1 -> dsync1/1, counter/1
  in2/1 -> din2/1
  din2/1 -> delay0/1(din)
  mux1/1 -> dmux1/1
  dmux1/1 -> delay1/1(din)
  delay0/1(dout) -> mux1/3, mux0/2
  dsync1/1 -> sync_delay/1
  shift/1 -> slice0/1
  dmux0/1 -> butterfly_direct/2(b)
  slice0/1 -> butterfly_direct/4(shift)
  delay1/1(dout) -> butterfly_direct/1(a)
  sync_delay/1 -> butterfly_direct/3(sync_in)
  of_in/1 -> logical1/2
  butterfly_direct/3(of) -> logical1/1
  butterfly_direct/1(a+bw) -> out1/1
  butterfly_direct/2(a-bw) -> out2/1
  logical1/1 -> of/1
  butterfly_direct/4(sync_out) -> sync_out/1

== system sparrow_albatros_spec_withgpio/fft_wideband_real/fft_direct/butterfly0_0/bus_add ==
  a : Inport
  b : Inport  Port=2
  a_debus : Subsystem  AncestorBlock=casper_library_flow_control/bus_expand  mask(bus_expand){mode=divisions of arbitrary size, outputNum=2, outputWidth=[24  24  24  24], outputBinaryPt=[17  17  17  17], outputArithmeticType=[1  1  1  1], show_format=on, outputToWorkspace=off, variablePrefix=, outputToModelAsWell=on}
      mask prompts: outputNum "Number of outputs:"; outputWidth "Output width:"; outputBinaryPt "Output binary point position:"; outputArithmeticType "Output arithmetic type (ufix=0, fix=1, bool=2):"; show_format "Print format string?"; outputToWorkspace "Output to workspace?"; variablePrefix "Variable name prefix:"; outputToModelAsWell "Output to model as well?"
      mask help:
      | Expands a 'bus' made using a bus_create or Xilinx
      | concat block.
      | The input will be divided into the specified number
      | of outputs with the specified arithmetic types.
      | Divisions are made from most significant bit.
      mask init: same as sparrow_albatros_spec_withgpio/bus_expand
      settings: AttributesFormatString=4 outputs: f24.17,f24.17,f24.17,f24.17,
      mask TypeOptions mode: divisions of equal size | divisions of arbitrary size
      mask Callback mode: %bus_expand_callback();
      mask Callback outputWidth: %bus_expand_callback();
      mask Callback outputToWorkspace: %bus_expand_callback();
  addsub{1..4} (4 alike) : xbsIndex_r4/AddSub  mode=Addition  use_carryin=off  use_carryout=off  en=off  latency=1  precision=User Defined  arith_type="Signed  (2's comp)"  n_bits=26  bin_pt=17  quantization=Truncate  overflow=Wrap  use_behavioral_HDL=on  hw_selection=Fabric  pipelined=on  dbl_ovrd=off  block_type=addsub
  b_debus : Subsystem  AncestorBlock=casper_library_flow_control/bus_expand  mask(bus_expand){mode=divisions of arbitrary size, outputNum=2, outputWidth=[25  25  25  25], outputBinaryPt=[17  17  17  17], outputArithmeticType=[1  1  1  1], show_format=on, outputToWorkspace=off, variablePrefix=, outputToModelAsWell=on}
      mask prompts: outputNum "Number of outputs:"; outputWidth "Output width:"; outputBinaryPt "Output binary point position:"; outputArithmeticType "Output arithmetic type (ufix=0, fix=1, bool=2):"; show_format "Print format string?"; outputToWorkspace "Output to workspace?"; variablePrefix "Variable name prefix:"; outputToModelAsWell "Output to model as well?"
      mask help:
      | Expands a 'bus' made using a bus_create or Xilinx
      | concat block.
      | The input will be divided into the specified number
      | of outputs with the specified arithmetic types.
      | Divisions are made from most significant bit.
      mask init: same as sparrow_albatros_spec_withgpio/bus_expand
      settings: AttributesFormatString=4 outputs: f25.17,f25.17,f25.17,f25.17,
      mask TypeOptions mode: divisions of equal size | divisions of arbitrary size
      mask Callback mode: %bus_expand_callback();
      mask Callback outputWidth: %bus_expand_callback();
      mask Callback outputToWorkspace: %bus_expand_callback();
  op_bussify : Subsystem  AncestorBlock=casper_library_flow_control/bus_create  mask(bus_create){inputNum=4}
      mask prompts: inputNum "Number of inputs:"
      mask init:
      | bus_create_init(gcb,...
      |     'inputNum', inputNum);
  dout : Outport
  wires:
  a/1 -> a_debus/1(bus_in)
  b/1 -> b_debus/1(bus_in)
  a_debus/1(msb_out4) -> addsub1/1
  b_debus/1(msb_out4) -> addsub1/2
  a_debus/2(out3) -> addsub2/1
  b_debus/2(out3) -> addsub2/2
  a_debus/3(out2) -> addsub3/1
  b_debus/3(out2) -> addsub3/2
  a_debus/4(lsb_out1) -> addsub4/1
  b_debus/4(lsb_out1) -> addsub4/2
  addsub1/1 -> op_bussify/1(in1)
  addsub2/1 -> op_bussify/2(in2)
  addsub3/1 -> op_bussify/3(in3)
  addsub4/1 -> op_bussify/4(in4)
  op_bussify/1(bus_out) -> dout/1
